simulink model "XTHERM02_reference"  (R2025a)
settings: Solver=FixedStepDiscrete  StartTime=0  StopTime=3600  FixedStep=1  RelTol=1e-3
undefined symbols (not defined in the file): ambient_temperature, cabin_internal_gain, cabin_temperature_setpoint, capacity_event_time, component_heat_load, component_heat_step_fraction, component_temperature_limit, compressor_capacity_loss, heat_step_time, refrigerant_capacity, solar_irradiance
settings Model: Creator=SimuVerity Contributors  LastModifiedBy=SimuVerity Contributors

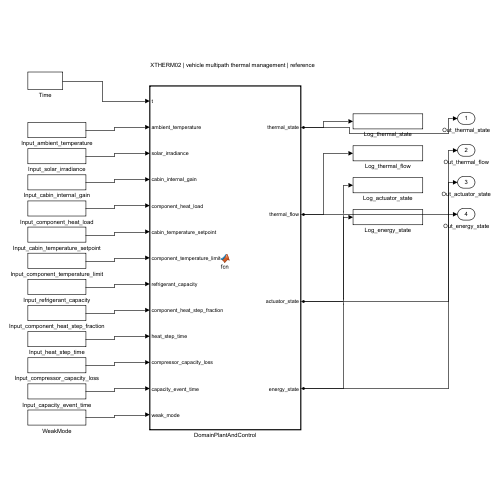
[thumbnail: Simulink's stored preview of the top-level diagram]
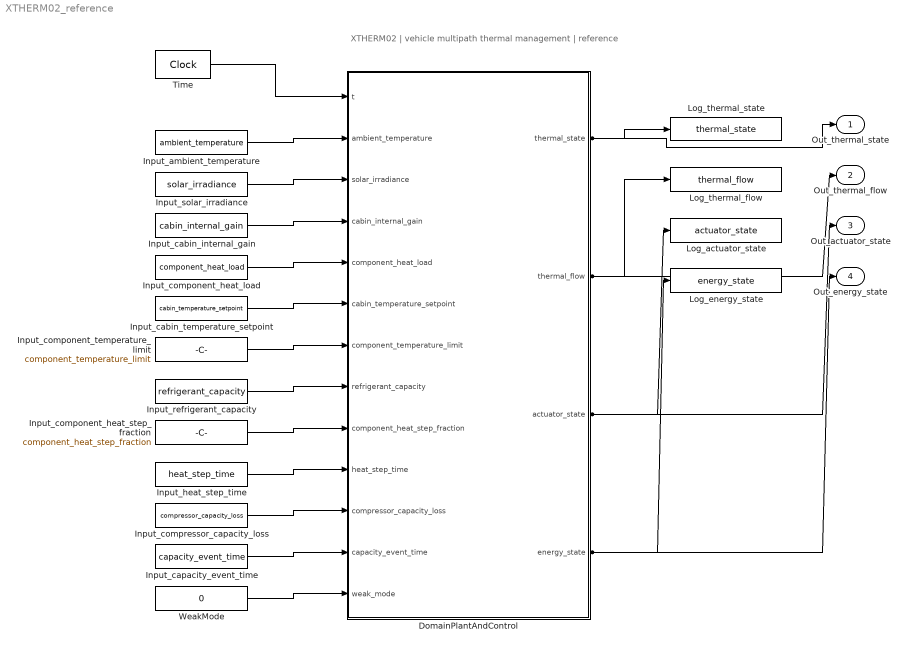
== system XTHERM02_reference ==
  note: XTHERM02 | vehicle multipath thermal management | reference
  DomainPlantAndControl : MATLAB Function  TreatAsAtomicUnit=on
  Input_ambient_temperature : Constant  Value=ambient_temperature
  Input_cabin_internal_gain : Constant  Value=cabin_internal_gain
  Input_cabin_temperature_setpoint : Constant  Value=cabin_temperature_setpoint
  Input_capacity_event_time : Constant  Value=capacity_event_time
  Input_component_heat_load : Constant  Value=component_heat_load
  Input_component_heat_step_fraction : Constant  Value=component_heat_step_fraction
  Input_component_temperature_limit : Constant  Value=component_temperature_limit
  Input_compressor_capacity_loss : Constant  Value=compressor_capacity_loss
  Input_heat_step_time : Constant  Value=heat_step_time
  Input_refrigerant_capacity : Constant  Value=refrigerant_capacity
  Input_solar_irradiance : Constant  Value=solar_irradiance
  Log_actuator_state : ToWorkspace  VariableName=actuator_state  SaveFormat=Timeseries  SampleTime=-1
  Log_energy_state : ToWorkspace  VariableName=energy_state  SaveFormat=Timeseries  SampleTime=-1
  Log_thermal_flow : ToWorkspace  VariableName=thermal_flow  SaveFormat=Timeseries  SampleTime=-1
  Log_thermal_state : ToWorkspace  VariableName=thermal_state  SaveFormat=Timeseries  SampleTime=-1
  Time : DigitalClock
  WeakMode : Constant  Value=0
  Out_thermal_state : Outport
  Out_thermal_flow : Outport  Port=2
  Out_actuator_state : Outport  Port=3
  Out_energy_state : Outport  Port=4
  wires:
  Time/1 -> DomainPlantAndControl/1(t)
  Input_ambient_temperature/1 -> DomainPlantAndControl/2(ambient_temperature)
  Input_solar_irradiance/1 -> DomainPlantAndControl/3(solar_irradiance)
  Input_cabin_internal_gain/1 -> DomainPlantAndControl/4(cabin_internal_gain)
  Input_component_heat_load/1 -> DomainPlantAndControl/5(component_heat_load)
  Input_cabin_temperature_setpoint/1 -> DomainPlantAndControl/6(cabin_temperature_setpoint)
  Input_component_temperature_limit/1 -> DomainPlantAndControl/7(component_temperature_limit)
  Input_refrigerant_capacity/1 -> DomainPlantAndControl/8(refrigerant_capacity)
  Input_component_heat_step_fraction/1 -> DomainPlantAndControl/9(component_heat_step_fraction)
  Input_heat_step_time/1 -> DomainPlantAndControl/10(heat_step_time)
  Input_compressor_capacity_loss/1 -> DomainPlantAndControl/11(compressor_capacity_loss)
  Input_capacity_event_time/1 -> DomainPlantAndControl/12(capacity_event_time)
  WeakMode/1 -> DomainPlantAndControl/13(weak_mode)
  DomainPlantAndControl/1(thermal_state) -> Log_thermal_state/1, Out_thermal_state/1
  DomainPlantAndControl/2(thermal_flow) -> Log_thermal_flow/1, Out_thermal_flow/1
  DomainPlantAndControl/3(actuator_state) -> Log_actuator_state/1, Out_actuator_state/1
  DomainPlantAndControl/4(energy_state) -> Log_energy_state/1, Out_energy_state/1

== matlab function XTHERM02_reference/DomainPlantAndControl ==
  data: t input; thermal_state output; ambient_temperature input; solar_irradiance input; cabin_internal_gain input; component_heat_load input; cabin_temperature_setpoint input; component_temperature_limit input; refrigerant_capacity input; component_heat_step_fraction input; heat_step_time input; compressor_capacity_loss input; capacity_event_time input; weak_mode input; thermal_flow output; actuator_state output; energy_state output
function [thermal_state,thermal_flow,actuator_state,energy_state] = fcn(t,ambient_temperature,solar_irradiance,cabin_internal_gain,component_heat_load,cabin_temperature_setpoint,component_temperature_limit,refrigerant_capacity,component_heat_step_fraction,heat_step_time,compressor_capacity_loss,capacity_event_time,weak_mode)
%#codegen
persistent Tcab Tmass Tcomp Tcool zCab zComp eComp ePump eBlower ePTC
dt=1; Ccab=6.0e5; Cmass=4.0e6; Ccomp=1.1e6; Ccool=1.6e6;
if isempty(Tcab) || t<0.5
    Tcab=ambient_temperature; Tmass=ambient_temperature;
    Tcomp=ambient_temperature; Tcool=ambient_temperature;
    zCab=0; zComp=0; eComp=0; ePump=0; eBlower=0; ePTC=0;
end
heatEvent=(t>=heat_step_time && t<heat_step_time+600);
capacityEvent=(t>=capacity_event_time && t<capacity_event_time+450);
qGeneration=component_heat_load*(1+component_heat_step_fraction*double(heatEvent));
availableCapacity=refrigerant_capacity*(1-compressor_capacity_loss*double(capacityEvent));
qCabinGain=cabin_internal_gain+3.0*solar_irradiance;
qAmbientCabin=105*(ambient_temperature-Tcab);
qAmbientMass=65*(ambient_temperature-Tmass);
qMassCabin=160*(Tmass-Tcab);
if weak_mode<0.5
    coolError=max(Tcab-cabin_temperature_setpoint,0);
    componentError=max(Tcomp-(component_temperature_limit-3),0);
    heatError=max(cabin_temperature_setpoint-Tcab,0);
    zCab=min(max(0.998*zCab+coolError*dt,0),18000);
    zComp=min(max(0.998*zComp+componentError*dt,0),18000);
    cabinFeedforward=max(qAmbientCabin+qMassCabin+qCabinGain,0);
    coolantPumpCommand=min(max(0.22+0.58*qGeneration/max(refrigerant_capacity,1)+0.10*componentError,0),1);
    radiatorBypass=double(Tcool<=ambient_temperature+0.5);
    radiatorEstimate=max((1-radiatorBypass)*(90+720*coolantPumpCommand)*(Tcool-ambient_temperature),0);
    cabinDemand=max(0,cabinFeedforward+2600*coolError+24*zCab);
    componentDemand=max(0,max(qGeneration-radiatorEstimate,0)+2400*componentError+20*zComp);
    totalDemand=cabinDemand+componentDemand;
    if totalDemand>1
        evaporatorAllocation=cabinDemand/totalDemand;
        chillerAllocation=componentDemand/totalDemand;
    else
        evaporatorAllocation=0; chillerAllocation=0;
    end
    compressorCommand=min(max(totalDemand/max(availableCapacity,1),0),1);
    coolantPumpCommand=max(coolantPumpCommand,min(max(0.12+0.70*componentDemand/max(availableCapacity,1),0),1));
    cabinBlowerCommand=min(max(0.10+0.75*cabinDemand/max(availableCapacity,1),0),1);
    ptcPower=min(max(2200*heatError,0),8000);
else
    % Weak baseline: fixed cooling allocation and weak open-loop actuation.
    compressorCommand=0.55;
    evaporatorAllocation=0.55; chillerAllocation=0.45;
    coolantPumpCommand=0.32; cabinBlowerCommand=0.45;
    radiatorBypass=double(ambient_temperature>290);
    ptcPower=min(max(420*(cabin_temperature_setpoint-ambient_temperature),0),2600);
end
totalCooling=availableCapacity*compressorCommand;
qEvaporator=totalCooling*evaporatorAllocation;
qChiller=totalCooling*chillerAllocation;
coolantMassFlow=0.35*coolantPumpCommand;
qComponentCoolant=(140+900*coolantPumpCommand)*(Tcomp-Tcool);
qRadiator=(1-radiatorBypass)*(90+720*coolantPumpCommand)*(Tcool-ambient_temperature);
cop=min(max(4.4-0.055*max(ambient_temperature-298.15,0),1.5),6);
compressorPower=totalCooling/cop;
pumpPower=220*coolantPumpCommand^3;
blowerPower=420*cabinBlowerCommand^3;
qPTC=ptcPower;
qCondenser=qEvaporator+qChiller+compressorPower;
dTcab=(qAmbientCabin+qMassCabin+qCabinGain+qPTC-qEvaporator)/Ccab;
dTmass=(qAmbientMass-qMassCabin)/Cmass;
dTcomp=(qGeneration-qComponentCoolant)/Ccomp;
dTcool=(qComponentCoolant-qChiller-qRadiator)/Ccool;
Tcab=Tcab+dt*dTcab; Tmass=Tmass+dt*dTmass;
Tcomp=Tcomp+dt*dTcomp; Tcool=Tcool+dt*dTcool;
eComp=eComp+dt*compressorPower/3.6e6;
ePump=ePump+dt*pumpPower/3.6e6;
eBlower=eBlower+dt*blowerPower/3.6e6;
ePTC=ePTC+dt*ptcPower/3.6e6;
thermal_state=[Tcab,Tmass,Tcomp,Tcool];
thermal_flow=[qAmbientCabin,qAmbientMass,qMassCabin,qCabinGain,qPTC,qEvaporator,qGeneration,qComponentCoolant,qChiller,qRadiator,qCondenser];
actuator_state=[compressorCommand,availableCapacity,evaporatorAllocation,chillerAllocation,coolantPumpCommand,coolantMassFlow,cabinBlowerCommand,radiatorBypass,compressorPower,pumpPower,blowerPower,ptcPower];
energy_state=[eComp,ePump,eBlower,ePTC];
end
